simulink subsystem "adrc_harness"  (R2026a)
settings: Solver=VariableStepAuto
undefined symbols (not defined in the file): ADC_Emulated_conversion_factor, ballscrew_travel_per_force, ballscrew_travel_per_rad, Bm, DiscIntNeverNeededParam, dspblkCoreblockFVToolHelper, excitation, gcbh, J, L, loadcell_bias, loadcell_offset, PsiM, PWMVoltage, r, rated_capacity, RT, sensitivity, Shunt_Amp_Offset, spring_constant, Ts_sim, VoltagetoADCValue
libraries: simulink x4
settings Model: Creator=drew  LastModifiedBy=Drew

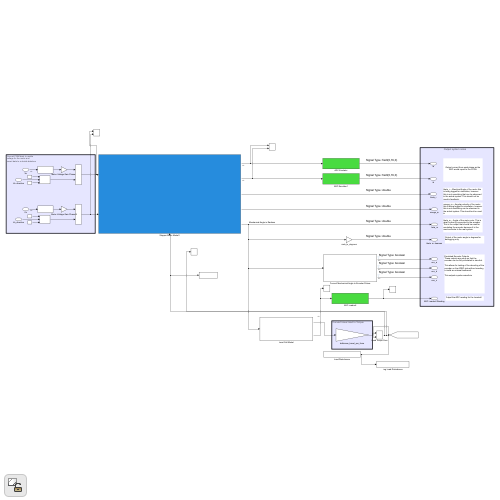
[thumbnail: Simulink's stored preview of the top-level diagram]
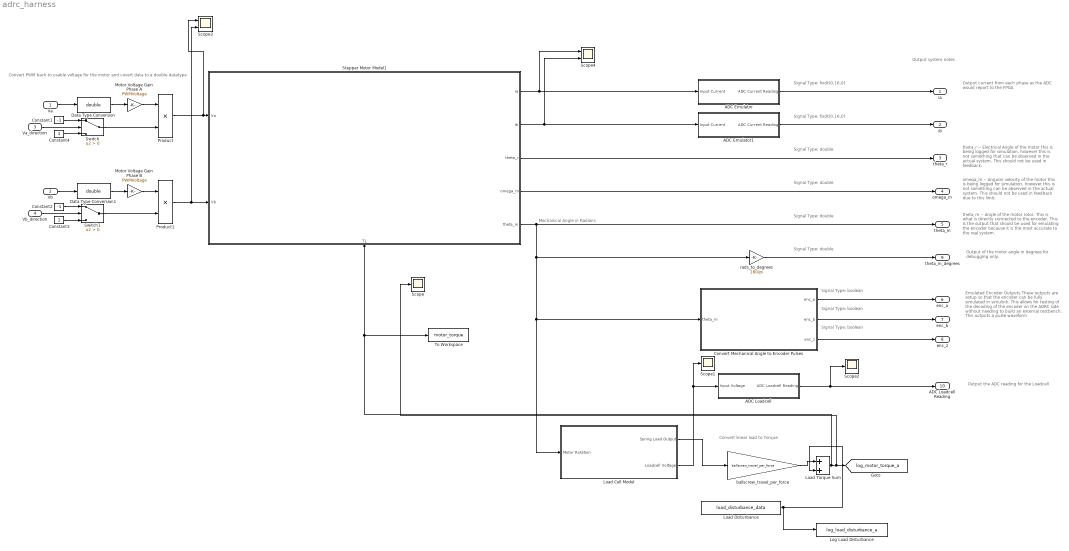
== system adrc_harness ==
  note: Convert linear load to Torque
  note: Signal Type: fixdt(0,16,0)
  note: Output of the motor angle in degrees for debugging only.
  note: omega_m -- Angular velocity of the motor
      | this is being logged for simulation, however
      | this is not something can be observed in
      | the actual system. This should not be used in
      | feedback due to this limit.
  note: Output current from each phase as the ADC would report to the FPGA
  note: theta_r -- Electrical Angle of the motor this
      | is being logged for simulation, however
      | this is not something that can be observed in the actual system. This should not be used in feedback.
  note: Output system notes
  note: Emulated Encoder Outputs
      | These outputs are setup so that the encoder can be fully simulated in simulink.
      |
      | This allows for testing of the decoding of the encoder on the ADRC side without needing to build an external testbench.
      |
      | This outputs a pulse waveform
  note: theta_m -- Angle of the motor rotor. This is what is directly connected to the encoder. This is the output that should be used for emulating the encoder because it is the most accurate to the real system.
  note: Convert PWM back to usable
      | voltage for the motor and
      | covert data to a double datatype
  note: Mechanical Angle in Radians
  note: Signal Type: fixdt(0,16,0)
  note: Signal Type: double
  note: Signal Type: double
  note: Signal Type: double
  note: Signal Type: double
  note: Signal Type: boolean
  note: Signal Type: boolean
  note: Signal Type: boolean
  note: Output the ADC reading for the Loadcell
  Va : Inport  OutDataTypeStr=boolean
  Vb : Inport  Port=2  OutDataTypeStr=boolean
  Va_direction : Inport  Port=3  OutDataTypeStr=boolean
  Vb_direction : Inport  Port=4  OutDataTypeStr=boolean
  ADC Emulator : Subsystem
  ADC Emulator1 : Subsystem
  ADC Loadcell : Subsystem
  Constant1 : Constant  Value=-1
  Constant2 : Constant  Value=-1
  Constant3 : Constant
  Constant4 : Constant
  Convert Mechanical Angle to Encoder Pulses : Subsystem
  Data Type Conversion : DataTypeConversion  OutDataTypeStr=double  SaturateOnIntegerOverflow=off  RndMeth=Floor
  Data Type Conversion1 : DataTypeConversion  OutDataTypeStr=double  SaturateOnIntegerOverflow=off  RndMeth=Floor
  Load Cell Model : Subsystem
  Load Disturbance : FromWorkspace  VariableName=load_disturbance_data  SampleTime=Ts_sim  Interpolate=off  ZeroCross=off  OutputAfterFinalValue=Holding final value
  Load Torque Sum : Sum
  Log Load Disturbance : ToWorkspace  VariableName=log_load_disturbance_a  SaveFormat=Timeseries  SampleTime=-1
      settings: Decimation=4000
  Motor Voltage Gain Phase A : Gain  Gain=PWMVoltage  ParamDataTypeStr=fixdt(1,16,8)  OutDataTypeStr=double
  Motor Voltage Gain Phase B : Gain  Gain=PWMVoltage  ParamDataTypeStr=fixdt(1,16,8)  OutDataTypeStr=double
  Product : Product
  Product1 : Product
  Scope : Scope
      settings: Title=Torque Load  ActiveDisplayYMinimum=-4.2407427932736113  ActiveDisplayYMaximum=4.0019633554117675  DataLoggingVariableName=ScopeData13
  Scope1 : Scope
      settings: ActiveDisplayYMinimum=-1.277986563252786E-10  ActiveDisplayYMaximum=1.1918161337435596E-9  DataLoggingVariableName=ScopeData14
  Scope2 : Scope
      settings: ActiveDisplayYMinimum=-1  ActiveDisplayYMaximum=3.9451219512195124  DataLoggingVariableName=ScopeData15
  Scope3 : Scope  NumInputPorts=2
      settings: Title=Actual Motor Voltages  ActiveDisplayYMinimum=-60  ActiveDisplayYMaximum=60  DataLoggingVariableName=ScopeData16
  Scope4 : Scope  NumInputPorts=2
      settings: Title=Actual Motor Currents  ActiveDisplayYMinimum=-3.75  ActiveDisplayYMaximum=3.75  DataLoggingVariableName=ScopeData17
  Stepper Motor Model1 : Subsystem
      settings: PortSchema="{\"entries\":[{\"content\":{\"sides\":[{\"content\":{\"connectorIds\":[\"In1\",\"In2\"]},\"type\":\"ConnectorPlacement.EquallySpacedRectSide\",\"uuid\":\"7511ab9d-0094-43d3-89f5-b2e49e4d50e0\"},{\"content\":{\"connectorIds\":[\"Out1\",\"Out2\",\"Out3\",\"Out4\",\"Out5\"],\"side\":\"RIGHT\"},\"type\":\"ConnectorPlacement.EquallySpacedRectSide\",\"uuid\":\"5cafba49-3cee-44c9-9e06-ed2832ee26a6\"},{\"content\":{\"side\":\"TOP\"},\"type\":\"ConnectorPlacement.EquallySpacedRectSide\",\"uuid\":\"e1ebdc11-237c-4bc0-9693-1fb398d141dc\"},{\"content\":{\"connectorIds\":[\"In3\"],\"side\":\"BOTTOM\"},\"type\":\"ConnectorPlacement.EquallySpacedRectSide\",\"uuid\":\"77cfc723-2a88-4b2a-9385-6805b8336786\"}]},\"type\":\"ConnectorPlacement.EquallySpacedConnector\",\"uuid\":\"1cbcd7b4-f556-40e4-9539-0630fd1e1098\"}],\"packageUris\":[\"http://schema.mathworks.com/mf0/Connector/R2020b\"],\"version\":\"1.0\"}"
  Switch : Switch  Criteria=u2 > Threshold  SaturateOnIntegerOverflow=off  InputSameDT=off
  Switch1 : Switch  Criteria=u2 > Threshold  SaturateOnIntegerOverflow=off  InputSameDT=off
  To Workspace : ToWorkspace  VariableName=motor_torque  SaveFormat=Timeseries  SampleTime=-1
      settings: Decimation=4000
  ballscrew_travel_per_force : Gain  Gain=ballscrew_travel_per_force
  rads_to_degrees : Gain  Gain=180/pi  OutDataTypeStr=double
  ia : Outport  OutDataTypeStr=uint16
  ib : Outport  Port=2  OutDataTypeStr=uint16
  theta_r : Outport  Port=3
  omega_m : Outport  Port=4
  theta_m : Outport  Port=5
  enc_a : Outport  Port=6
  enc_b : Outport  Port=7
  enc_z : Outport  Port=8
  theta_m_degrees : Outport  Port=9
  ADC Loadcell Reading : Outport  Port=10
  tag scope: log_motor_torque_a=global
  wires:
  ADC Emulator/1(ADC Current Reading) -> ia/1
  ADC Emulator1/1(ADC Current Reading) -> ib/1
  Stepper Motor Model1/3(theta_r) -> theta_r/1
  Stepper Motor Model1/4(omega_m) -> omega_m/1
  Stepper Motor Model1/5(theta_m) -> theta_m/1, rads_to_degrees/1, Convert Mechanical Angle to Encoder Pulses/1(theta_m), Load Cell Model/1("Motor Rotation ")
  rads_to_degrees/1 -> theta_m_degrees/1
  Motor Voltage Gain Phase A/1 -> Product/1
  Motor Voltage Gain Phase B/1 -> Product1/1
  Data Type Conversion1/1 -> Motor Voltage Gain Phase B/1
  Data Type Conversion/1 -> Motor Voltage Gain Phase A/1
  Vb/1 -> Data Type Conversion1/1
  Va/1 -> Data Type Conversion/1
  Convert Mechanical Angle to Encoder Pulses/1(enc_a) -> enc_a/1
  Convert Mechanical Angle to Encoder Pulses/2(enc_b) -> enc_b/1
  Convert Mechanical Angle to Encoder Pulses/3(enc_z) -> enc_z/1
  Stepper Motor Model1/1(Ia) -> ADC Emulator/1(Input Current), Scope4/1
  Stepper Motor Model1/2(Ib) -> ADC Emulator1/1(Input Current), Scope4/2
  Product/1 -> Stepper Motor Model1/1(Va), Scope3/1
  Switch/1 -> Product/2
  Va_direction/1 -> Switch/2
  Constant4/1 -> Switch/3
  Constant1/1 -> Switch/1
  Constant2/1 -> Switch1/1
  Constant3/1 -> Switch1/3
  Vb_direction/1 -> Switch1/2
  Product1/1 -> Stepper Motor Model1/2(Vb), Scope3/2
  Switch1/1 -> Product1/2
  Load Cell Model/1(Spring Load Output) -> ballscrew_travel_per_force/1
  ADC Loadcell/1(ADC Loadcell Reading) -> ADC Loadcell Reading/1, Scope2/1
  Load Cell Model/2(Loadcell Voltage) -> ADC Loadcell/1(Input Voltage), Scope1/1
  ballscrew_travel_per_force/1 -> Load Torque Sum/1
  Load Disturbance/1 -> Load Torque Sum/2, Log Load Disturbance/1
  Load Torque Sum/1 -> Stepper Motor Model1/3(TL), To Workspace/1, Scope/1, [log_motor_torque_a]

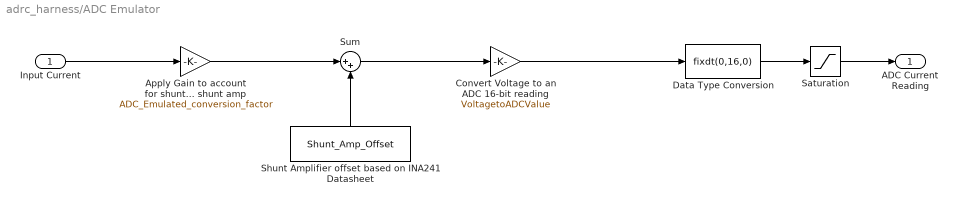
== system adrc_harness/ADC Emulator ==
  Input Current : Inport
  Apply Gain to account for shunt resistor and shunt amp : Gain  Gain=ADC_Emulated_conversion_factor  ParamDataTypeStr=fixdt(1,16,8)  RndMeth=Round
  Convert Voltage to an ADC 16-bit reading : Gain  Gain=VoltagetoADCValue  ParamDataTypeStr=int16  OutMin=[0]  OutMax=[4095]  OutDataTypeStr=double  RndMeth=Round  SaturateOnIntegerOverflow=on
  Data Type Conversion : DataTypeConversion  OutDataTypeStr=fixdt(0,16,0)  RndMeth=Round
  Saturation : Saturate  UpperLimit=65535  LowerLimit=0
  Shunt Amplifier offset based on INA241 Datasheet : Constant  Value=Shunt_Amp_Offset  OutDataTypeStr=double
  Sum : Sum  Inputs=|++  OutDataTypeStr=Inherit: Inherit via back propagation
  ADC Current Reading : Outport
  wires:
  Apply Gain to account for shunt resistor and shunt amp/1 -> Sum/1
  Shunt Amplifier offset based on INA241 Datasheet/1 -> Sum/2
  Input Current/1 -> Apply Gain to account for shunt resistor and shunt amp/1
  Sum/1 -> Convert Voltage to an ADC 16-bit reading/1
  Convert Voltage to an ADC 16-bit reading/1 -> Data Type Conversion/1
  Data Type Conversion/1 -> Saturation/1
  Saturation/1 -> ADC Current Reading/1

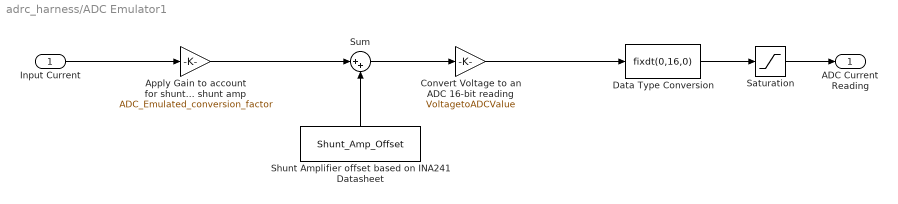
== system adrc_harness/ADC Emulator1 ==
  Input Current : Inport
  Apply Gain to account for shunt resistor and shunt amp : Gain  Gain=ADC_Emulated_conversion_factor  ParamDataTypeStr=fixdt(1,16,8)  RndMeth=Round
  Convert Voltage to an ADC 16-bit reading : Gain  Gain=VoltagetoADCValue  ParamDataTypeStr=int16  OutMin=[0]  OutMax=[4095]  OutDataTypeStr=double  RndMeth=Round  SaturateOnIntegerOverflow=on
  Data Type Conversion : DataTypeConversion  OutDataTypeStr=fixdt(0,16,0)  RndMeth=Round
  Saturation : Saturate  UpperLimit=65535  LowerLimit=0
  Shunt Amplifier offset based on INA241 Datasheet : Constant  Value=Shunt_Amp_Offset  OutDataTypeStr=fixdt(1,16,8)
  Sum : Sum  Inputs=|++  OutDataTypeStr=Inherit: Inherit via back propagation
  ADC Current Reading : Outport
  wires:
  Apply Gain to account for shunt resistor and shunt amp/1 -> Sum/1
  Shunt Amplifier offset based on INA241 Datasheet/1 -> Sum/2
  Input Current/1 -> Apply Gain to account for shunt resistor and shunt amp/1
  Sum/1 -> Convert Voltage to an ADC 16-bit reading/1
  Convert Voltage to an ADC 16-bit reading/1 -> Data Type Conversion/1
  Data Type Conversion/1 -> Saturation/1
  Saturation/1 -> ADC Current Reading/1

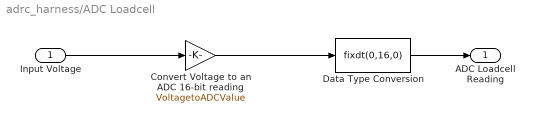
== system adrc_harness/ADC Loadcell ==
  Input Voltage : Inport
  Convert Voltage to an ADC 16-bit reading : Gain  Gain=VoltagetoADCValue  ParamDataTypeStr=int16  OutMin=[0]  OutMax=[4095]  OutDataTypeStr=double  SaturateOnIntegerOverflow=on
  Data Type Conversion : DataTypeConversion  OutDataTypeStr=fixdt(0,16,0)  RndMeth=Nearest
  ADC Loadcell Reading : Outport
  wires:
  Convert Voltage to an ADC 16-bit reading/1 -> Data Type Conversion/1
  Data Type Conversion/1 -> ADC Loadcell Reading/1
  Input Voltage/1 -> Convert Voltage to an ADC 16-bit reading/1

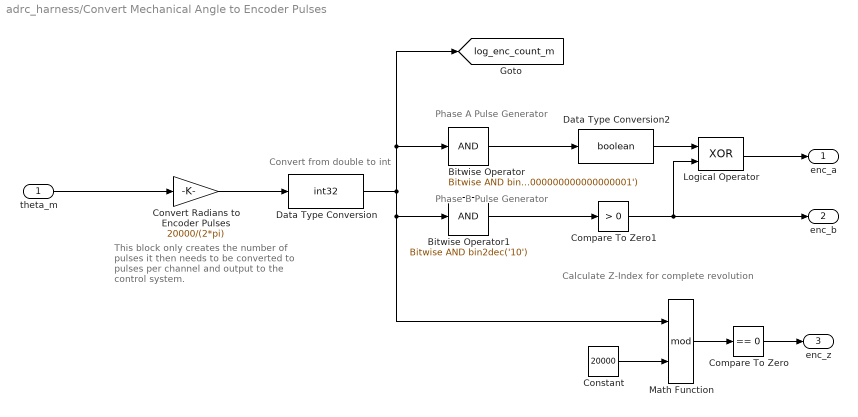
== system adrc_harness/Convert Mechanical Angle to Encoder Pulses ==
  note: Calculate Z-Index for complete revolution
  note: Phase B Pulse Generator
  note: Phase A Pulse Generator
  note: Convert from double to int
  note: This block only creates the number of pulses it then needs to be converted to pulses per channel and output to the control system.
  theta_m : Inport  OutDataTypeStr=double
  Bitwise Operator : simulink/Logic and Bit Operations/Bitwise Operator  logicop=AND  UseBitMask=on  BitMask=bin2dec('00000000000000000000000000000001')  BitMaskRealWorld=Stored Integer
  Bitwise Operator1 : simulink/Logic and Bit Operations/Bitwise Operator  logicop=AND  UseBitMask=on  BitMask=bin2dec('10')  BitMaskRealWorld=Stored Integer
  Compare To Zero : simulink/Logic and Bit Operations/Compare To Zero  relop===  OutDataTypeStr=boolean
  Compare To Zero1 : simulink/Logic and Bit Operations/Compare To Zero  relop=>  OutDataTypeStr=boolean
  Constant : Constant  Value=20000  OutDataTypeStr=int32
  Convert Radians to Encoder Pulses : Gain  Gain=20000/(2*pi)  OutDataTypeStr=double
  Data Type Conversion : DataTypeConversion  OutDataTypeStr=int32  SaturateOnIntegerOverflow=off  RndMeth=Floor
  Data Type Conversion2 : DataTypeConversion  OutDataTypeStr=boolean  SaturateOnIntegerOverflow=off  RndMeth=Floor
  Logical Operator : Logic  Operator=XOR  AllPortsSameDT=off  OutDataTypeStr=boolean
  Math Function : Math  Operator=mod
  enc_a : Outport  OutDataTypeStr=boolean
  enc_b : Outport  Port=2  OutDataTypeStr=boolean
  enc_z : Outport  Port=3  OutDataTypeStr=boolean
  tag scope: log_enc_count_m=global
  wires:
  Data Type Conversion2/1 -> Logical Operator/1
  Logical Operator/1 -> enc_a/1
  Math Function/1 -> Compare To Zero/1
  Constant/1 -> Math Function/2
  Compare To Zero1/1 -> enc_b/1, Logical Operator/2
  Bitwise Operator1/1 -> Compare To Zero1/1
  Compare To Zero/1 -> enc_z/1
  Convert Radians to Encoder Pulses/1 -> Data Type Conversion/1
  Bitwise Operator/1 -> Data Type Conversion2/1
  Data Type Conversion/1 -> Bitwise Operator/1, [log_enc_count_m], Bitwise Operator1/1, Math Function/1
  theta_m/1 -> Convert Radians to Encoder Pulses/1

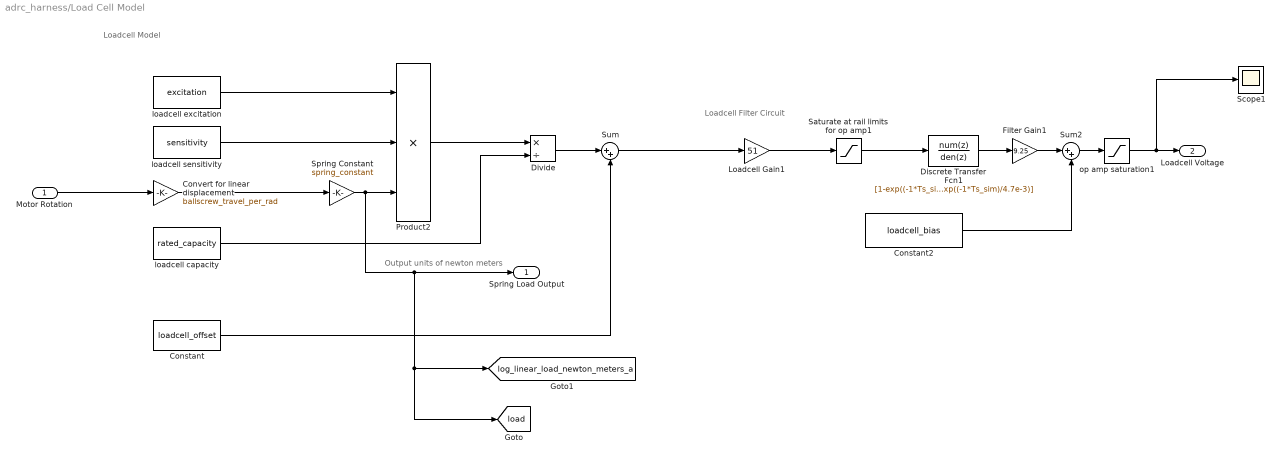
== system adrc_harness/Load Cell Model ==
  note: Loadcell Filter Circuit
  note: Loadcell Model
  note: Output units of newton meters
  "Motor Rotation " : Inport
  Constant : Constant  Value=loadcell_offset
  Constant2 : Constant  Value=loadcell_bias
  Convert for linear displacement : Gain  Gain=ballscrew_travel_per_rad
  Discrete Transfer Fcn1 : DiscreteTransferFcn  LoadFcn=dspblkCoreblockFVToolHelper(gcbh,'load');  Numerator=[1-exp((-1*Ts_sim)/4.7e-3)]  Denominator=[1 -exp((-1*Ts_sim)/4.7e-3)]
      settings: CopyFcn=dspblkCoreblockFVToolHelper(gcbh,'copy');  DeleteFcn=dspblkCoreblockFVToolHelper(gcbh,'close');  ModelCloseFcn=dspblkCoreblockFVToolHelper(gcbh,'close');  PreSaveFcn=dspblkCoreblockFVToolHelper(gcbh,'presave');  PostSaveFcn=dspblkCoreblockFVToolHelper(gcbh,'postsave');  CloseFcn=dspblkCoreblockFVToolHelper(gcbh,'close');
  Divide : Product  Inputs=*/
  Filter Gain1 : Gain  Gain=9.25
  Loadcell Gain1 : Gain  Gain=51
  Product2 : Product  Inputs=3
  Saturate at rail limits for op amp1 : Saturate  UpperLimit=4.72  LowerLimit=-5+0.35
  Scope1 : Scope
      settings: ActiveDisplayYMinimum=-1  ActiveDisplayYMaximum=1  DataLoggingVariableName=ScopeData22
  Spring Constant : Gain  Gain=spring_constant
  Sum : Sum  Inputs=|++
  Sum2 : Sum  Inputs=|++
  loadcell capacity : Constant  Value=rated_capacity
  loadcell excitation : Constant  Value=excitation
  loadcell sensitivity : Constant  Value=sensitivity
  op amp saturation1 : Saturate  UpperLimit=5-0.2  LowerLimit=0
  Spring Load Output : Outport
  Loadcell Voltage : Outport  Port=2
  tag scope: load=global, log_linear_load_newton_meters_a=global
  wires:
  Loadcell Gain1/1 -> Saturate at rail limits for op amp1/1
  Sum/1 -> Loadcell Gain1/1
  Discrete Transfer Fcn1/1 -> Filter Gain1/1
  op amp saturation1/1 -> Loadcell Voltage/1, Scope1/1
  Saturate at rail limits for op amp1/1 -> Discrete Transfer Fcn1/1
  Constant2/1 -> Sum2/2
  Filter Gain1/1 -> Sum2/1
  Sum2/1 -> op amp saturation1/1
  Convert for linear displacement/1 -> Spring Constant/1
  Constant/1 -> Sum/2
  Product2/1 -> Divide/1
  loadcell capacity/1 -> Divide/2
  loadcell sensitivity/1 -> Product2/2
  Divide/1 -> Sum/1
  Spring Constant/1 -> Product2/3, Spring Load Output/1, [load], [log_linear_load_newton_meters_a]
  "Motor Rotation "/1 -> Convert for linear displacement/1
  loadcell excitation/1 -> Product2/1

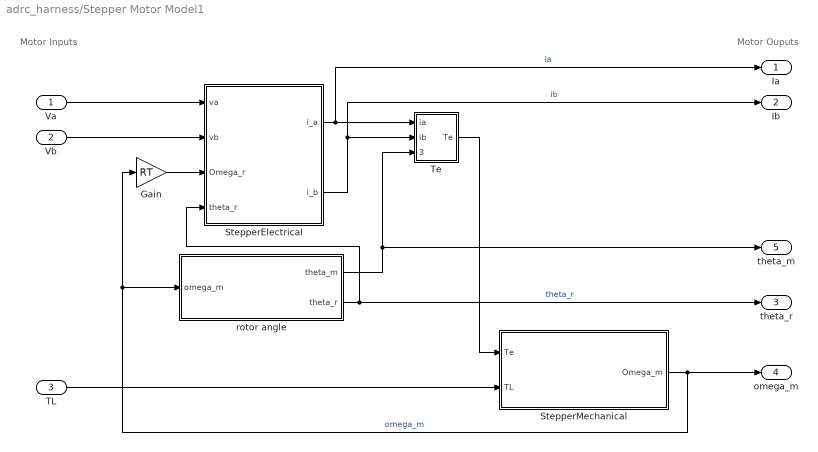
== system adrc_harness/Stepper Motor Model1 ==
  note: Motor Ouputs
  note: Motor Inputs
  Va : Inport  OutDataTypeStr=double
  Vb : Inport  Port=2  OutDataTypeStr=double
  TL : Inport  Port=3
  Gain : Gain  Gain=RT  OutDataTypeStr=double
  StepperElectrical : Subsystem
  StepperMechanical : Subsystem
  Te : Subsystem
  rotor angle : Subsystem
  Ia : Outport  OutDataTypeStr=double
  Ib : Outport  Port=2  OutDataTypeStr=double
  theta_r : Outport  Port=3  OutDataTypeStr=double
  omega_m : Outport  Port=4  OutDataTypeStr=double
  theta_m : Outport  Port=5  OutDataTypeStr=double
  wires:
  TL/1 -> StepperMechanical/2(TL)
  Vb/1 -> StepperElectrical/2(vb)
  rotor angle/2(theta_r) -> theta_r/1, StepperElectrical/4(theta_r)  "theta_r"
  StepperElectrical/1(i_a) -> Te/1(ia), Ia/1  "ia"
  Gain/1 -> StepperElectrical/3(Omega_r)
  rotor angle/1(theta_m) -> Te/3(theta_m), theta_m/1
  Va/1 -> StepperElectrical/1(va)
  StepperMechanical/1(Omega_m) -> Gain/1, rotor angle/1(omega_m), omega_m/1  "omega_m"
  StepperElectrical/2(i_b) -> Te/2(ib), Ib/1  "ib"
  Te/1(Te) -> StepperMechanical/1(Te)

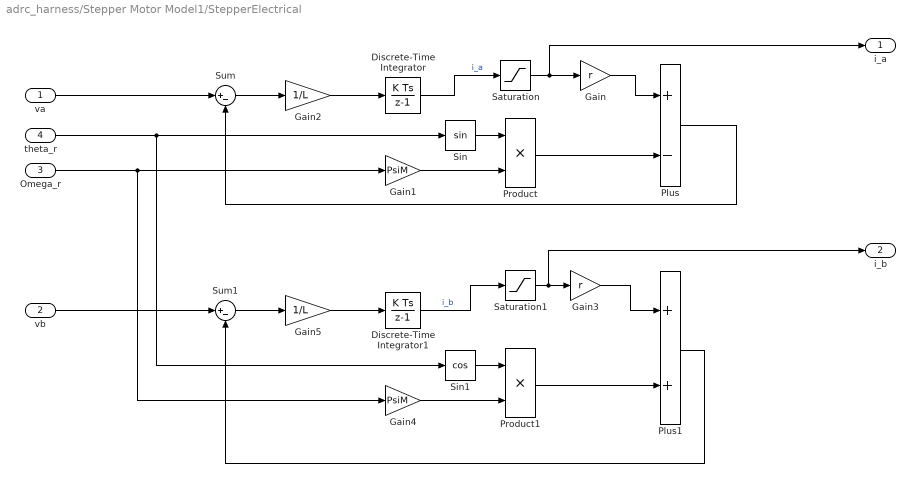
== system adrc_harness/Stepper Motor Model1/StepperElectrical ==
  va : Inport  OutDataTypeStr=double
  vb : Inport  Port=2  OutDataTypeStr=double
  Omega_r : Inport  Port=3  OutDataTypeStr=double
  theta_r : Inport  Port=4  OutDataTypeStr=double
  Discrete-Time Integrator : DiscreteIntegrator  SampleTime=Ts_sim  OutDataTypeStr=double  SaturateOnIntegerOverflow=on  ICPrevOutput=DiscIntNeverNeededParam  ICPrevScaledInput=DiscIntNeverNeededParam
  Discrete-Time Integrator1 : DiscreteIntegrator  SampleTime=Ts_sim  OutDataTypeStr=double  SaturateOnIntegerOverflow=on  ICPrevOutput=DiscIntNeverNeededParam  ICPrevScaledInput=DiscIntNeverNeededParam
  Gain : Gain  Gain=r  ParamDataTypeStr=double  OutDataTypeStr=double
  Gain1 : Gain  Gain=PsiM  OutDataTypeStr=double
  Gain2 : Gain  Gain=1/L  OutDataTypeStr=double
  Gain3 : Gain  Gain=r  OutDataTypeStr=double
  Gain4 : Gain  Gain=PsiM  OutDataTypeStr=double
  Gain5 : Gain  Gain=1/L  OutDataTypeStr=double
  Plus : Sum  Inputs=+-  OutDataTypeStr=double
  Plus1 : Sum  OutDataTypeStr=double
  Product : Product  OutDataTypeStr=double
  Product1 : Product  OutDataTypeStr=double
  Saturation : Saturate  UpperLimit=4.243  LowerLimit=-4.243
  Saturation1 : Saturate  UpperLimit=4.243  LowerLimit=-4.243
  Sin : Trigonometry
  Sin1 : Trigonometry  Operator=cos
  Sum : Sum  Inputs=|+-  OutDataTypeStr=double
  Sum1 : Sum  Inputs=|+-  OutDataTypeStr=double
  i_a : Outport  OutDataTypeStr=double
  i_b : Outport  Port=2  OutDataTypeStr=double
  wires:
  Saturation1/1 -> Gain3/1, i_b/1
  Saturation/1 -> Gain/1, i_a/1
  Discrete-Time Integrator/1 -> Saturation/1  "i_a"
  Gain/1 -> Plus/1
  Gain2/1 -> Discrete-Time Integrator/1
  Omega_r/1 -> Gain4/1, Gain1/1
  Sum/1 -> Gain2/1
  Product/1 -> Plus/2
  Gain5/1 -> Discrete-Time Integrator1/1
  Gain4/1 -> Product1/2
  Plus/1 -> Sum/2
  Discrete-Time Integrator1/1 -> Saturation1/1  "i_b"
  Sin/1 -> Product/1
  Sum1/1 -> Gain5/1
  Product1/1 -> Plus1/2
  Gain3/1 -> Plus1/1
  vb/1 -> Sum1/1
  Plus1/1 -> Sum1/2
  Gain1/1 -> Product/2
  Sin1/1 -> Product1/1
  theta_r/1 -> Sin1/1, Sin/1
  va/1 -> Sum/1

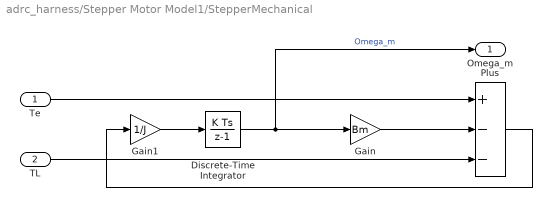
== system adrc_harness/Stepper Motor Model1/StepperMechanical ==
  Te : Inport  OutDataTypeStr=double
  TL : Inport  Port=2  OutDataTypeStr=double
  Discrete-Time Integrator : DiscreteIntegrator  SampleTime=Ts_sim  OutDataTypeStr=double  SaturateOnIntegerOverflow=on  ICPrevOutput=DiscIntNeverNeededParam  ICPrevScaledInput=DiscIntNeverNeededParam
  Gain : Gain  Gain=Bm  OutDataTypeStr=double
  Gain1 : Gain  Gain=1/J  OutDataTypeStr=double
  Plus : Sum  Inputs=+--  OutDataTypeStr=double
  Omega_m : Outport  OutDataTypeStr=double
  wires:
  Plus/1 -> Gain1/1
  Gain1/1 -> Discrete-Time Integrator/1
  TL/1 -> Plus/3
  Gain/1 -> Plus/2
  Discrete-Time Integrator/1 -> Omega_m/1, Gain/1  "Omega_m"
  Te/1 -> Plus/1

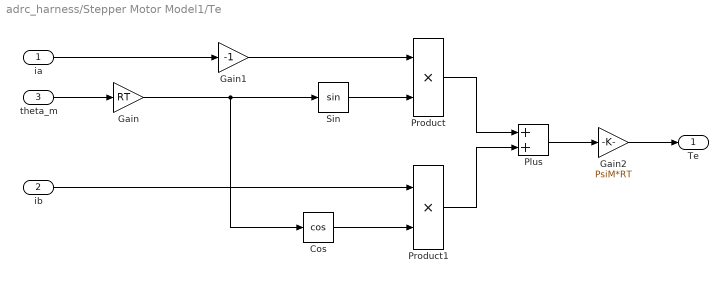
== system adrc_harness/Stepper Motor Model1/Te ==
  ia : Inport  OutDataTypeStr=double
  ib : Inport  Port=2  OutDataTypeStr=double
  theta_m : Inport  Port=3  OutDataTypeStr=double
  Cos : Trigonometry  Operator=cos
  Gain : Gain  Gain=RT  OutDataTypeStr=double
  Gain1 : Gain  Gain=-1  OutDataTypeStr=double
  Gain2 : Gain  Gain=PsiM*RT  OutDataTypeStr=double
  Plus : Sum  OutDataTypeStr=double
  Product : Product  OutDataTypeStr=double
  Product1 : Product  OutDataTypeStr=double
  Sin : Trigonometry
  Te : Outport  OutDataTypeStr=double
  wires:
  Gain/1 -> Sin/1, Cos/1
  theta_m/1 -> Gain/1
  Plus/1 -> Gain2/1
  Gain2/1 -> Te/1
  Product/1 -> Plus/1
  ia/1 -> Gain1/1
  Product1/1 -> Plus/2
  ib/1 -> Product1/1
  Cos/1 -> Product1/2
  Sin/1 -> Product/2
  Gain1/1 -> Product/1

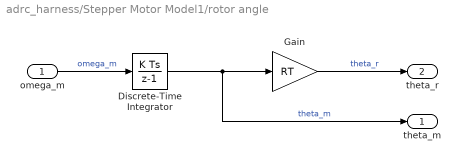
== system adrc_harness/Stepper Motor Model1/rotor angle ==
  omega_m : Inport  OutDataTypeStr=double
  Discrete-Time Integrator : DiscreteIntegrator  SampleTime=Ts_sim  OutDataTypeStr=double  SaturateOnIntegerOverflow=on  ICPrevOutput=DiscIntNeverNeededParam  ICPrevScaledInput=DiscIntNeverNeededParam
  Gain : Gain  Gain=RT  OutDataTypeStr=double
  theta_m : Outport  OutDataTypeStr=double
  theta_r : Outport  Port=2  OutDataTypeStr=double
  wires:
  omega_m/1 -> Discrete-Time Integrator/1  "omega_m"
  Gain/1 -> theta_r/1  "theta_r"
  Discrete-Time Integrator/1 -> theta_m/1, Gain/1  "theta_m"
